simulink model "ASM_Traffic_new"  (R2024a)
settings: Solver=ode1  StartTime=SIM.tstart.v  StopTime=SIM.tend.v  FixedStep=SIM.StepSize.v  RelTol=1e-3
PostLoadFcn:
  | if any(exist('dsrtsu_mdlpostloadfcn', 'file') ~= 0), dsrtsu_mdlpostloadfcn('Execute', bdroot); end
  | try, asm_mdl_postloadfcn(bdroot, 'UpdateModel', 3600); catch, disp(lasterr); end,
InitFcn:
  | , if any(exist('rtifpga_mdlclblib', 'file') ~= 0), rtifpga_mdlclblib('Init', bdroot); end,
  | , if any(exist('dsmpb_private', 'file') ~= 0), dsmpb_private('dsmpb_mdlclblib', 'Init', bdroot); end,
undefined symbols (not defined in the file): _to_, a0b2, ASM_BrakeHydraulics_DemoSystems, ASM_VehicleDynamics_DemoSystems, b98103fe8ad365046cd0, BrakeCircuit, CPT, Crankshaft, DiscIntNeverNeededParam, dsmsi, FinalDriveAssembly, MDL, ModeSignals, Pos_BrakePedal_Maneuver, rad, RefSignals, s_to_rpm, SIM, SoftECU, Suspension, Tire, Transmission
libraries: ASM_Traffic_lib x135, simulink x100, ASM_Utils_lib x77, ASM_VehicleDynamics_lib x70, ASM_Environment_lib x22, dsmpblib x20, dsmsilib x15, MDLD_Utils_lib x10, ASM_BrakeHydraulics_lib x3
(part 26 of 63)

== system ASM_Traffic_new/Environment/Sensors/PlantModel/Collision_Sensor ==
  Enable_Init[0Off|1On] : Inport
  Enable[0Off|1On] : Inport  Port=2
  Traffic_Signals : Inport  Port=3
  Interface_In : Inport  Port=4
  Road_Signals : Inport  Port=5
  Maneuver_Signals : Inport  Port=6
  ASMSignalCollector : Subsystem
  Bus Selector : BusSelector  OutputSignals=Plant.Traffic_Signals_toEnvironment.v_Fellows[x;y;z][km|h],Plant.Traffic_Signals_toEnvironment.w_Fellows[x;y;z][deg|s]
  Bus Selector1 : BusSelector  OutputSignals=ExternalModel.Pos_Vehicle_CoorSys_E[x;y;z][m],ExternalModel.Angle_Vehicle_CoorSys_E[x;y;z][deg],ExternalModel.v_x_Vehicle_CoG[km|h],ExternalModel.v_y_Vehicle_CoG[km|h],ExternalModel.YawRate_Vehicle_CoG[deg|s]
  Bus Selector2 : BusSelector  OutputSignals=Plant.ObjectParameters.FellowParameters.TrafficObject_Type_Fellows[],Plant.ObjectParameters.TrafficObjects.TrafficObject_Type_Data[],Plant.ObjectParameters.DiscreteObjects.DiscreteObject_Data[]
  Bus Selector3 : BusSelector  OutputSignals=Plant.TrafficObject_Data[]
  Bus Selector4 : BusSelector  OutputSignals=Plant.Traffic_Signals_toEnvironment
  Bus Selector5 : BusSelector  OutputSignals=Plant.ManeuverScheduler.Info.ManeuverTime[s],Plant.ManeuverScheduler.Parameters.Object_Type_ID[]
  Bus Selector6 : BusSelector  OutputSignals=Info.Flag_Sensor_Init_Ready[0|1]  OutputAsBus=on
  Bus Selector7 : BusSelector  OutputSignals=Plant.Traffic_Signals_toEnvironment.Flag_FellowUsed[0|1]
  Bus Selector8 : BusSelector  OutputSignals=Plant.ObjectParameters.TrafficObjects.TrafficObjectsState[],Plant.ObjectParameters.DiscreteObjects.DiscreteObjectsState[]
  COLLISION_SENSOR : ASM_Traffic_lib/Sensors/Collision_Sensor/COLLISION_SENSOR  Tag=ASM_SUBCOMPONENT  Sw_Sensor_Enable=MDL.Traffic.Sensors.CollisionSensor.Sw_Sensor_Enable  Sw_Detection_Mode=MDL.Traffic.Sensors.CollisionSensor.Sw_Detection_Mode  Const_Collisions_OutputDimension=MDL.Traffic.Sensors.CollisionSensor.Const_Sensor_Output_Dimension  ASMProperties=struct('Name','COLLISION_SENSOR','Version','5.0','Library','ASM_Traffic_lib')  ASMInstanceName=collision_sensor  ASMInstanceID=1
  Constant : Constant  Value=0
  Demux : Demux  Outputs=3
  Enable_Collision_Sensor : Subsystem
  ExternalUserData : Subsystem
  GetFellowPositionVector : Subsystem
  Mux : Mux  Inputs=3
  Mux1 : Mux  Inputs=2
  Mux2 : Mux  Inputs=2
  SensorsGotoTagVisiblity : GotoTagVisibility  GotoTag=ASMBUS_Traf_Sensors_Collision_Sensor_1
  Terminator : Terminator
  Terminator2 : Terminator
  Terminator3 : Terminator
  Sensor_Signals : Outport  VectorParamsAs1DForOutWhenUnconnected=off
  tag scope: ASMBUS_Traf_Sensors_Collision_Sensor_1=scoped
  wires:
  Bus Selector7/1 -> COLLISION_SENSOR/9  "<Flag_FellowUsed[0|1]>"
  GetFellowPositionVector/2(Angle_Fellows[deg]) -> COLLISION_SENSOR/11
  GetFellowPositionVector/1(Pos_Fellows_MainPnt_CoorSys_E[x;y;z][m]) -> COLLISION_SENSOR/10
  Bus Selector4/1 -> GetFellowPositionVector/1(<FellowPositions>)  "<Traffic_Signals_toEnvironment>"
  Bus Selector6/1 -> Terminator3/1
  COLLISION_SENSOR/2 -> Bus Selector6/1, Sensor_Signals/1
  Enable_Init[0Off|1On]/1 -> COLLISION_SENSOR/1
  ExternalUserData/1(Flag_CollsionSensor_Parameters_Used_External[0|1]) -> COLLISION_SENSOR/14
  ExternalUserData/4(Pos_y_CollisionObj_Custom_RefPnt_External[m]) -> Mux1/2
  ExternalUserData/3(Pos_x_CollisionObj_Custom_RefPnt_External[m]) -> Mux1/1
  Bus Selector/1 -> COLLISION_SENSOR/12  "<v_Fellows[x;y;z][km|h]>"
  Bus Selector/2 -> Demux/1  "<w_Fellows[x;y;z][deg|s]>"
  Demux/3 -> COLLISION_SENSOR/13
  Demux/1 -> Terminator/1
  Demux/2 -> Terminator2/1
  Constant/1 -> Mux/3
  Bus Selector5/1 -> COLLISION_SENSOR/7  "<ManeuverTime[s]>"
  Bus Selector5/2 -> COLLISION_SENSOR/8  "<Object_Type_ID[]>"
  Maneuver_Signals/1 -> Bus Selector5/1
  Mux/1 -> COLLISION_SENSOR/5
  COLLISION_SENSOR/1 -> [ASMBUS_Traf_Sensors_Collision_Sensor_1]
  Bus Selector3/1 -> COLLISION_SENSOR/20  "<TrafficObject_Data[]>"
  Bus Selector2/3 -> COLLISION_SENSOR/19  "<DiscreteObject_Data[]>"
  Bus Selector2/2 -> COLLISION_SENSOR/18  "<TrafficObject_Type_Data[]>"
  Bus Selector2/1 -> COLLISION_SENSOR/17  "<TrafficObject_Type_Fellows[]>"
  Mux1/1 -> COLLISION_SENSOR/16
  ExternalUserData/2(TrafficObject_Type_CollisionObj_External[]) -> COLLISION_SENSOR/15
  Bus Selector1/5 -> COLLISION_SENSOR/6  "<YawRate_Vehicle_CoG[deg|s]>"
  Bus Selector1/4 -> Mux/2  "<v_y_Vehicle_CoG[km|h]>"
  Bus Selector1/3 -> Mux/1  "<v_x_Vehicle_CoG[km|h]>"
  Bus Selector1/2 -> COLLISION_SENSOR/4  "<Angle_Vehicle_CoorSys_E[x;y;z][deg]>"
  Bus Selector1/1 -> COLLISION_SENSOR/3  "<Pos_Vehicle_CoorSys_E[x;y;z][m]>"
  Enable_Collision_Sensor/1(Enable_Out[0Off|1On]) -> COLLISION_SENSOR/2
  Enable[0Off|1On]/1 -> Enable_Collision_Sensor/1(Enable_In[0Off|1On])
  Interface_In/1 -> Bus Selector1/1
  Road_Signals/1 -> Bus Selector3/1
  Bus Selector8/2 -> Mux2/2  "<DiscreteObjectsState[]>"
  Mux2/1 -> COLLISION_SENSOR/21
  Bus Selector8/1 -> Mux2/1  "<TrafficObjectsState[]>"
  Traffic_Signals/1 -> Bus Selector7/1, Bus Selector4/1, Bus Selector2/1, Bus Selector8/1, Bus Selector/1

== system ASM_Traffic_new/Environment/Sensors/PlantModel/Line_Sensor ==
  Enable[0Off|1On] : Inport
  Interface_In : Inport  Port=2
  Road_Signals : Inport  Port=3
  Maneuver_Signals : Inport  Port=4
  ASMSignalCollector : Subsystem
  Bus Selector15 : BusSelector  OutputSignals=ExternalModel.Pos_Vehicle_CoorSys_E[x;y;z][m],ExternalModel.Angle_Vehicle_CoorSys_E[x;y;z][deg]
  Bus Selector2 : BusSelector  OutputSignals=Plant.Road_Info.Line_Sensor_Data
  Bus Selector5 : BusSelector  OutputSignals=Plant.ManeuverScheduler.MdlControl.Reset_VehicleStates[0|1],Plant.ManeuverScheduler.Info.ManeuverState[],Plant.ManeuverScheduler.InitialVehStates.Route_Id_Init[],Plant.ManeuverScheduler.InitialVehStates.Route_Direction_Init[]
  Bus Selector6 : BusSelector  OutputSignals=Plant.Road_ASMVeh.s_Veh_Road[m],Plant.Road_Info.d_Veh_Ref_Line[m]
  Demux : Demux  Outputs=3
  Demux1 : Demux  Outputs=3
  Enable_Line_Sensor : Subsystem
  LINE_SENSOR : ASM_Traffic_lib/Sensors/Line_Sensor/LINE_SENSOR  Tag=ASM_SUBCOMPONENT  Const_Length_Sensor_Range=MDL.Traffic.Sensors.LineSensor.Const_Length_Sensor_Range  Const_Num_Lines_Per_Side_Max=MDL.Traffic.Sensors.LineSensor.Const_Num_Lines_Per_Side_Max  Const_Dist_Road_Sample_Pnts=MDL.Traffic.Sensors.LineSensor.Const_Dist_Road_Sample_Pnts  Const_Road_Lane_Output_Dimension=MDL.Traffic.Sensors.LineSensor.Const_Road_Lane_Output_Dimension  Const_Road_Shape_Line_Output_Dimension=MDL.Traffic.Sensors.LineSensor.Const_Road_Shape_Line_Output_Dimension  Const_Road_Shape_ContObj_Output_Dimension=MDL.Traffic.Sensors.LineSensor.Const_Road_Shape_ContObj_Output_Dimension  Const_Junction_Border_Output_Dimension=MDL.Traffic.Sensors.LineSensor.Const_Junction_Border_Output_Dimension  Const_Junction_Shape_Line_Output_Dimension=MDL.Traffic.Sensors.LineSensor.Const_Junction_Shape_Line_Output_Dimension  Const_Junction_Shape_ContObj_Output_Dimension=MDL.Traffic.Sensors.LineSensor.Const_Junction_Shape_ContObj_Output_Dimension  Sw_Sensor_Enable=MDL.Traffic.Sensors.LineSensor.Sw_Sensor_Enable  ASMProperties=struct('Name','LINE_SENSOR','Version','8.0','Library','ASM_Traffic_lib')  ASMInstanceName=line_sensor  ASMInstanceID=1
  SensorsGotoTagVisiblity : GotoTagVisibility  GotoTag=ASMBUS_Traf_Sensors_Line_Sensor_1
  Terminator17 : Terminator
  Terminator18 : Terminator
  Terminator19 : Terminator
  Sensor_Signals : Outport  VectorParamsAs1DForOutWhenUnconnected=off
  tag scope: ASMBUS_Traf_Sensors_Line_Sensor_1=scoped
  wires:
  Enable_Line_Sensor/1(Enable_Out[0Off|1On]) -> LINE_SENSOR/1
  Bus Selector6/2 -> LINE_SENSOR/8  "<d_Veh_Ref_Line[m]>"
  Interface_In/1 -> Bus Selector15/1
  Bus Selector6/1 -> LINE_SENSOR/7  "<s_Veh_Road[m]>"
  Road_Signals/1 -> Bus Selector2/1, Bus Selector6/1
  Bus Selector5/4 -> LINE_SENSOR/6  "<Route_Direction_Init[]>"
  Bus Selector5/3 -> LINE_SENSOR/5  "<Route_Id_Init[]>"
  Bus Selector5/2 -> LINE_SENSOR/4  "<ManeuverState[]>"
  Bus Selector5/1 -> LINE_SENSOR/3  "<Reset_VehicleStates[0|1]>"
  Maneuver_Signals/1 -> Bus Selector5/1
  Enable[0Off|1On]/1 -> Enable_Line_Sensor/1(Enable_In[0Off|1On])
  Bus Selector2/1 -> LINE_SENSOR/2  "<Line_Sensor_Data>"
  LINE_SENSOR/2 -> Sensor_Signals/1
  LINE_SENSOR/1 -> [ASMBUS_Traf_Sensors_Line_Sensor_1]
  Demux/1 -> Terminator19/1
  Demux1/3 -> Terminator18/1
  Bus Selector15/2 -> Demux/1  "<Angle_Vehicle_CoorSys_E[x;y;z][deg]>"
  Demux/2 -> Terminator17/1
  Bus Selector15/1 -> Demux1/1  "<Pos_Vehicle_CoorSys_E[x;y;z][m]>"
  Demux1/1 -> LINE_SENSOR/9
  Demux1/2 -> LINE_SENSOR/10
  Demux/3 -> LINE_SENSOR/11

== system ASM_Traffic_new/Environment/Sensors/PlantModel/Object_Sensor_2D ==
  Enable_Init[0Off|1On] : Inport
  Enable[0Off|1On] : Inport  Port=2
  Traffic_Signals : Inport  Port=3
  Interface_In : Inport  Port=4
  Road_Signals : Inport  Port=5
  ASMSignalCollector : Subsystem
  Enable_Object_Sensor_2D : Subsystem
  ObjectData : Subsystem
  ScheduleAndCalculateSensor : Subsystem
  SensorMapping : Subsystem
  SensorParameters : Subsystem
  SensorsGotoTagVisiblity1 : GotoTagVisibility  GotoTag=ASMBUS_Environment_Traffic_2DObjSensor_ObjectData
  SensorsGotoTagVisiblity2 : GotoTagVisibility  GotoTag=ASMBUS_Environment_Traffic_SensorScheduler_ObjectSensor2D
  SensorsGotoTagVisiblity3 : GotoTagVisibility  GotoTag=ASMBUS_Environment_Traffic_2DObjSensor_Parameter
  SensorsGotoTagVisiblity4 : GotoTagVisibility  GotoTag=ASMBUS_Environment_Traffic_2DObjSensorCalc_Info
  SensorsGotoTagVisiblity5 : GotoTagVisibility  GotoTag=ASMBUS_Environment_Traffic_2DObjSensor_SensorSignals
  SensorsGotoTagVisiblity6 : GotoTagVisibility  GotoTag=ASMBUS_Environment_Traffic_SamplePulse_ObjectSensor2D
  Sensor_Signals : Outport  VectorParamsAs1DForOutWhenUnconnected=off
  Init_Ready[0Off|1On] : Outport  Port=2  VectorParamsAs1DForOutWhenUnconnected=off
  wires:
  ScheduleAndCalculateSensor/3(Init_Ready[0Off|1On]) -> Init_Ready[0Off|1On]/1
  Enable_Init[0Off|1On]/1 -> ScheduleAndCalculateSensor/1(Enable_Init[0Off|1On])
  Enable[0Off|1On]/1 -> Enable_Object_Sensor_2D/1(Enable_In[0Off|1On])
  Enable_Object_Sensor_2D/1(Enable_Out[0Off|1On]) -> SensorMapping/1(Enable[0Off|1On]), ScheduleAndCalculateSensor/3(Enable[0Off|1On])
  SensorMapping/1(Sensor_Signals) -> Sensor_Signals/1
  Interface_In/1 -> ScheduleAndCalculateSensor/5(Interface_In)
  Traffic_Signals/1 -> ScheduleAndCalculateSensor/4(Traffic_Signals), ObjectData/1(Traffic_Signals)
  Road_Signals/1 -> ScheduleAndCalculateSensor/6(Road_Signals), ObjectData/2(Road_Signals)
  ScheduleAndCalculateSensor/1(SensorMapping_Data[]) -> SensorMapping/2(SensorMapping_Data[])
  ScheduleAndCalculateSensor/2(SensorSignals) -> SensorMapping/3(SensorSignals)
  SensorParameters/1(Sensor_Data[]) -> ScheduleAndCalculateSensor/2(Sensor_Data[])

== system ASM_Traffic_new/Environment/Sensors/PlantModel/Object_Sensor_3D ==
  Enable_Init[0Off|1On] : Inport
  Enable[0Off|1On] : Inport  Port=2
  Traffic_Signals : Inport  Port=3
  Interface_In : Inport  Port=4
  Road_Signals : Inport  Port=5
  Sensor_Time_Base[s] : Inport  Port=6
  ASMSignalCollector : Subsystem
  CustomPoints : Subsystem
  Enable_Object_Sensor_3D : Subsystem
  ObjectData : Subsystem
  RadarEffects : Subsystem
  ScheduleAndCalculateSensor : Subsystem
  SensorMapping : Subsystem
  SensorParameters : Subsystem
  SensorsGotoTagVisiblity1 : GotoTagVisibility  GotoTag=ASMBUS_Environment_Traffic_3DObjSensor_CustomPoints
  SensorsGotoTagVisiblity10 : GotoTagVisibility  GotoTag=ASMBUS_Environment_Traffic_3DObjSensor2_Parameters
  SensorsGotoTagVisiblity11 : GotoTagVisibility  GotoTag=ASMBUS_Environment_Traffic_3DObjSensor3_Parameters
  SensorsGotoTagVisiblity2 : GotoTagVisibility  GotoTag=ASMBUS_Environment_Traffic_3DObjSensors_Boundingboxes
  SensorsGotoTagVisiblity3 : GotoTagVisibility  GotoTag=ASMBUS_Environment_Traffic_3DObjSensor_ObjectData
  SensorsGotoTagVisiblity4 : GotoTagVisibility  GotoTag=ASMBUS_Environment_Traffic_3DObjSensor_RadarEffects
  SensorsGotoTagVisiblity5 : GotoTagVisibility  GotoTag=ASMBUS_Environment_Traffic_SensorScheduler
  SensorsGotoTagVisiblity6 : GotoTagVisibility  GotoTag=ASMBUS_Environment_Traffic_SamplePulse
  SensorsGotoTagVisiblity7 : GotoTagVisibility  GotoTag=ASMBUS_Environment_Traffic_3DObjSensor_SensorSignals_Status
  SensorsGotoTagVisiblity8 : GotoTagVisibility  GotoTag=ASMBUS_Environment_Traffic_3DObjSensor_SensorSignals
  SensorsGotoTagVisiblity9 : GotoTagVisibility  GotoTag=ASMBUS_Environment_Traffic_3DObjSensor1_Parameters
  Sensor_Signals : Outport  VectorParamsAs1DForOutWhenUnconnected=off
  Init_Ready[0Off|1On] : Outport  Port=2  VectorParamsAs1DForOutWhenUnconnected=off
  wires:
  ScheduleAndCalculateSensor/3(SensorData[]) -> RadarEffects/4(SensorData[]), CustomPoints/3(SensorData[])
  ScheduleAndCalculateSensor/4(Angle_Vehicle_CoorSys_E_Sampled[x,y;z][deg]) -> RadarEffects/5(Angle_Vehicle_CoorSys_E[x;y;z][deg])
  ScheduleAndCalculateSensor/5(Pos_Vehicle_CoorSys_E_Sampled[x,y;z][m]) -> RadarEffects/6(Pos_Vehicle_CoorSys_E[x;y;z][m])
  Enable_Init[0Off|1On]/1 -> ScheduleAndCalculateSensor/1(Enable_Init[0Off|1On]), RadarEffects/1(Enable_Init[0Off|1On])
  ScheduleAndCalculateSensor/6(Init_Ready[0Off|1On]) -> Init_Ready[0Off|1On]/1
  Enable[0Off|1On]/1 -> Enable_Object_Sensor_3D/1(Enable_In[0Off|1On])
  Enable_Object_Sensor_3D/1(Enable_Out[0Off|1On]) -> ScheduleAndCalculateSensor/3(Enable[0Off|1On]), CustomPoints/1(Enable[0Off|1On]), RadarEffects/2(Enable[0Off|1On]), SensorMapping/1(Enable[0Off|1On])
  SensorMapping/1(Sensor_Signals) -> Sensor_Signals/1
  Interface_In/1 -> ScheduleAndCalculateSensor/5(Interface_In)
  SensorParameters/1(Sensor_Data[]) -> ScheduleAndCalculateSensor/2(Sensor_Data[])
  Traffic_Signals/1 -> ObjectData/1(Traffic_Signals), ScheduleAndCalculateSensor/4(Traffic_Signals)
  Road_Signals/1 -> ObjectData/2(Road_Signals), ScheduleAndCalculateSensor/6(Road_Signals)
  ScheduleAndCalculateSensor/1(SensorMapping_Data[]) -> CustomPoints/2(SensorMapping_Data[]), RadarEffects/3(SensorMapping_Data[]), SensorMapping/2(SensorMapping_Data[])
  ScheduleAndCalculateSensor/2(SensorSignals) -> SensorMapping/3(SensorSignals)
  Sensor_Time_Base[s]/1 -> ScheduleAndCalculateSensor/7(Sensor_Time_Base[s])

== system ASM_Traffic_new/Environment/Sensors/PlantModel/Sensors_Common_Signals ==
  In : Inport
  Init_Ready[0Off|1On] : Inport  Port=2
  Brake : RelationalOperator  Operator===  OutDataTypeStr=boolean  InputSameDT=off
  Bus Selector2 : BusSelector  OutputSignals=Traffic.Plant.ObjectParameters.DiscreteObjects.Flag_DiscreteObject_Init_Ready[0|1]
  Bus Selector7 : BusSelector  OutputSignals=Maneuver.Plant.ManeuverScheduler.Info.ManeuverState[]  OutputAsBus=on
  Constant : Constant  Value=3
  Constant1 : Constant  Value=4
  Data Type Conversion : DataTypeConversion  OutDataTypeStr=double  SaturateOnIntegerOverflow=off  RndMeth=Floor
  Enable_Scheduling : Subsystem
  Logical Operator : Logic  Operator=OR  AllPortsSameDT=off  OutDataTypeStr=boolean
  Logical Operator1 : Logic  AllPortsSameDT=off
  Maneuver_Start : Subsystem
  Memory : UnitDelay  SampleTime=-1  HasFrameUpgradeWarning=on
  Run : RelationalOperator  Operator===  OutDataTypeStr=boolean  InputSameDT=off
  Sensor_Init_Trigger : Subsystem
  Sensor_Time_Base : Subsystem
  SignalCollector : Subsystem
  ASMSignalBus : Outport  VectorParamsAs1DForOutWhenUnconnected=off
  Enable_Init[0Off|1On] : Outport  Port=2  VectorParamsAs1DForOutWhenUnconnected=off
  Enable_Sensor_Scheduling_By_Init_Ready[0Off|1On] : Outport  Port=3  VectorParamsAs1DForOutWhenUnconnected=off
  Enable_Sensor_Scheduling[0Off|1On] : Outport  Port=4  VectorParamsAs1DForOutWhenUnconnected=off
  Sensor_Time_Base[s] : Outport  Port=5
  wires:
  Bus Selector2/1 -> Sensor_Init_Trigger/1(DiscreteObjects_Data_Valid[])  "<Flag_DiscreteObject_Init_Ready[0|1]>"
  Sensor_Init_Trigger/1(Ctrl) -> Enable_Init[0Off|1On]/1
  Init_Ready[0Off|1On]/1 -> Memory/1, SignalCollector/3(Init_Ready[0Off|1On])
  Memory/1 -> Logical Operator1/1
  Logical Operator1/1 -> Enable_Sensor_Scheduling_By_Init_Ready[0Off|1On]/1
  Enable_Scheduling/1(Enable_Out[0Off|1On]) -> Logical Operator1/2, Enable_Sensor_Scheduling[0Off|1On]/1
  Data Type Conversion/1 -> Enable_Scheduling/1(Enable_In[0Off|1On]), SignalCollector/2(Enable_SensorScheduling[0Off|1On])
  SignalCollector/1(ASMSignalBus) -> ASMSignalBus/1
  Brake/1 -> Logical Operator/2
  Bus Selector7/1 -> Brake/1, Run/1
  Constant1/1 -> Brake/2
  Run/1 -> Logical Operator/1
  Constant/1 -> Run/2
  Maneuver_Start/1(ManeuverStart[s]) -> Sensor_Time_Base/2(ManeuverStart[s]), SignalCollector/1(ManeuverStart[s])
  In/1 -> Bus Selector2/1, Bus Selector7/1
  Logical Operator/1 -> Sensor_Time_Base/1(ManeuverState_Change[0|1]), Maneuver_Start/1(ManeuverState_Change[0|1]), Data Type Conversion/1
  Sensor_Time_Base/1(Sensor_Time_Base[s]) -> Sensor_Time_Base[s]/1

== system ASM_Traffic_new/Environment/Sensors/PlantModel/Traffic_Sign_Sensor ==
  Interface_In : Inport
  Traffic_Signals : Inport  Port=2
  Road_Signals : Inport  Port=3
  Objects_DataStream_Signals : Inport  Port=4
  ASMSignalCollector : Subsystem
  Bus Selector1 : BusSelector  OutputSignals=ExternalModel.Pos_Vehicle_CoorSys_E[x;y;z][m],ExternalModel.Angle_Vehicle_CoorSys_E[x;y;z][deg]
  Bus Selector2 : BusSelector  OutputSignals=Plant.ObjectParameters.TrafficObjects.TrafficObject_Type_Data[]
  Bus Selector3 : BusSelector  OutputSignals=Plant.TrafficObject_Data[]
  Enable_Traffic_Sign_Sensor : Subsystem
  Mux : Mux  Inputs=6
  Objects_DataStreams : Subsystem
  SensorsGotoTagVisiblity : GotoTagVisibility  GotoTag=ASMBUS_Traf_Sensors_Traffic_Sign_Sensor_dyn_1_Parameters
  SensorsGotoTagVisiblity1 : GotoTagVisibility  GotoTag=ASMBUS_Traf_Sensors_dyn_Traffic_Sign_Sensor_1
  TRAFFIC_SIGN_SENSOR_DYNAMIC_CALCULATION : ASM_Traffic_lib/Sensors/Traffic_Sign_Sensor/TRAFFIC_SIGN_SENSOR_DYNAMIC_CALCULATION  Tag=ASM_SUBCOMPONENT  Const_Sensor_Output_Dimension=MDL.Traffic.Sensors.TrafficSignSensorDyn_Calculation.Const_Sensor_Output_Dimension  ASMProperties=struct('Name','TRAFFIC_SIGN_SENSOR_DYNAMIC_CALCULATION','Version','2.0','Library','ASM_Traffic_lib')  ASMInstanceName=traffic_sign_sensor_dynamic_calculation  ASMInstanceID=1
  TRAFFIC_SIGN_SENSOR_GEOMETRY_PARAMETERS : ASM_Traffic_lib/Sensors/Traffic_Sign_Sensor/TRAFFIC_SIGN_SENSOR_GEOMETRY_PARAMETERS  Tag=ASM_SUBCOMPONENT  Sensor_Enable=MDL.Traffic.Sensors.TrafficSignSensor_Geometry.Sw_Sensor_Enable  Pos_Sensor=MDL.Traffic.Sensors.TrafficSignSensor_Geometry.Const_Pos_Sensor_Apex_CoorSys_V  Angle_Orientation_Sensor=MDL.Traffic.Sensors.TrafficSignSensor_Geometry.Const_Angle_Orientation_Sensor_CoorSys_V  Length_ScopeZone=MDL.Traffic.Sensors.TrafficSignSensor_Geometry.Const_Length_ScopeZone  Angle_ScopeZone_Horizontal=MDL.Traffic.Sensors.TrafficSignSensor_Geometry.Const_Angle_ScopeZone_Horizontal  Angle_ScopeZone_Vertical=MDL.Traffic.Sensors.TrafficSignSensor_Geometry.Const_Angle_ScopeZone_Vertical  Angle_Sign_Orientation_Max=MDL.Traffic.Sensors.TrafficSignSensor_Geometry.Const_Angle_Sign_Orientation_Max  ASMProperties=struct('Name','TRAFFIC_SIGN_SENSOR_GEOMETRY_PARAMETERS','Version','2.0','Library','ASM_Traffic_lib')  ASMInstanceName=traffic_sign_sensor_geometry_parameters  ASMInstanceID=1
  Sensor_Signals : Outport  VectorParamsAs1DForOutWhenUnconnected=off
  tag scope: ASMBUS_Traf_Sensors_Traffic_Sign_Sensor_dyn_1_Parameters=scoped, ASMBUS_Traf_Sensors_dyn_Traffic_Sign_Sensor_1=scoped
  wires:
  Objects_DataStream_Signals/1 -> Objects_DataStreams/1(TrafficObjects_States_In[])
  Objects_DataStreams/1(TrafficObjects_States[]) -> TRAFFIC_SIGN_SENSOR_DYNAMIC_CALCULATION/7
  Bus Selector3/1 -> TRAFFIC_SIGN_SENSOR_DYNAMIC_CALCULATION/6  "<TrafficObject_Data[]>"
  Bus Selector2/1 -> TRAFFIC_SIGN_SENSOR_DYNAMIC_CALCULATION/5  "<TrafficObject_Type_Data[]>"
  Bus Selector1/2 -> TRAFFIC_SIGN_SENSOR_DYNAMIC_CALCULATION/4  "<Angle_Vehicle_CoorSys_E[x;y;z][deg]>"
  Bus Selector1/1 -> TRAFFIC_SIGN_SENSOR_DYNAMIC_CALCULATION/3  "<Pos_Vehicle_CoorSys_E[x;y;z][m]>"
  TRAFFIC_SIGN_SENSOR_DYNAMIC_CALCULATION/2 -> Sensor_Signals/1
  TRAFFIC_SIGN_SENSOR_DYNAMIC_CALCULATION/1 -> [ASMBUS_Traf_Sensors_dyn_Traffic_Sign_Sensor_1]
  Enable_Traffic_Sign_Sensor/1(Enable_Out[0Off|1On]) -> TRAFFIC_SIGN_SENSOR_DYNAMIC_CALCULATION/1
  TRAFFIC_SIGN_SENSOR_GEOMETRY_PARAMETERS/1 -> [ASMBUS_Traf_Sensors_Traffic_Sign_Sensor_dyn_1_Parameters]
  TRAFFIC_SIGN_SENSOR_GEOMETRY_PARAMETERS/2 -> Enable_Traffic_Sign_Sensor/1(Enable_In[0Off|1On])
  Mux/1 -> TRAFFIC_SIGN_SENSOR_DYNAMIC_CALCULATION/2
  TRAFFIC_SIGN_SENSOR_GEOMETRY_PARAMETERS/8 -> Mux/6
  TRAFFIC_SIGN_SENSOR_GEOMETRY_PARAMETERS/7 -> Mux/5
  TRAFFIC_SIGN_SENSOR_GEOMETRY_PARAMETERS/6 -> Mux/4
  TRAFFIC_SIGN_SENSOR_GEOMETRY_PARAMETERS/5 -> Mux/3
  TRAFFIC_SIGN_SENSOR_GEOMETRY_PARAMETERS/4 -> Mux/2
  TRAFFIC_SIGN_SENSOR_GEOMETRY_PARAMETERS/3 -> Mux/1
  Road_Signals/1 -> Bus Selector3/1
  Traffic_Signals/1 -> Bus Selector2/1
  Interface_In/1 -> Bus Selector1/1

== system ASM_Traffic_new/Environment/Sensors/UserInterface/ASMSignalBus_Plant ==
  In : Inport
  Terminator_1 : Terminator
  tag scope: ASMBUS_Environment_Traffic_Sensors=global
  wires:
  In/1 -> [ASMBUS_Environment_Traffic_Sensors]
  [ASMBUS_Environment_Traffic_Sensors] -> Terminator_1/1

== system ASM_Traffic_new/Environment/Sensors/UserInterface/DISP_Plant ==
  In : Inport
  Line_Sensor : Subsystem
  Object_Sensor_2D : Subsystem
  Object_Sensor_3D : Subsystem
  Traffic_Sign_Sensor : Subsystem
  wires:
  In/1 -> Line_Sensor/1(TrafficBus), Traffic_Sign_Sensor/1(TrafficBus), Object_Sensor_2D/1(TrafficBus), Object_Sensor_3D/1(TrafficBus)

== system ASM_Traffic_new/Environment/Sensors/UserInterface/PAR_Plant ==
  note: Control
  note: Inport colors:
  note: -------------
  note: Plant
  note: External Signals
  note: -------------
  note: -------------
  note: -------------
  note: User Interface
  In : Inport
  Constant : Constant
  Terminator1 : Terminator
  Out : Outport  VectorParamsAs1DForOutWhenUnconnected=off
  wires:
  Constant/1 -> Out/1  "UserInterface"
  In/1 -> Terminator1/1
